simulink subsystem "removeQuatZero"  (R2026a)
settings: Solver=VariableStepAuto
settings Model: Creator=maxhu  LastModifiedBy=maxhu

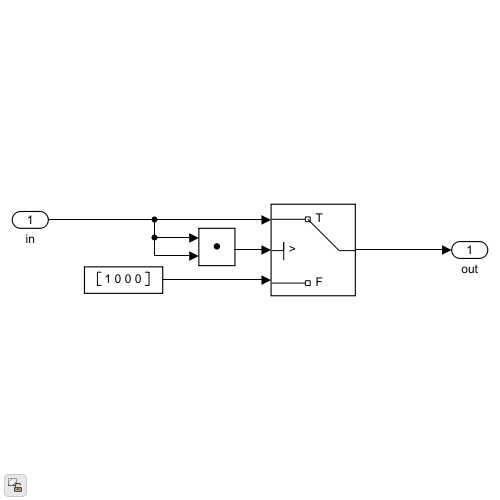
[thumbnail: Simulink's stored preview of the top-level diagram]
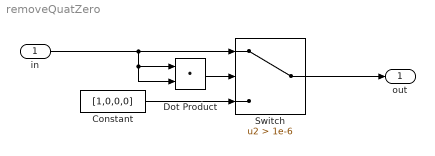
== system removeQuatZero ==
  in : Inport
  Constant : Constant  Value=[1,0,0,0]
  Dot Product : DotProduct  OutDataTypeStr=Inherit: Inherit via internal rule
  Switch : Switch  Criteria=u2 > Threshold  Threshold=1e-6  SaturateOnIntegerOverflow=off  InputSameDT=off
  out : Outport
  wires:
  Dot Product/1 -> Switch/2
  Switch/1 -> out/1
  Constant/1 -> Switch/3
  in/1 -> Switch/1, Dot Product/2, Dot Product/1
